simulink model "ASM_Traffic"  (R2026a)
settings: Solver=ode1  StartTime=SIM.tstart.v  StopTime=SIM.tend.v  FixedStep=SIM.StepSize.v
PostLoadFcn:
  | if any(exist('dsrtsu_mdlpostloadfcn', 'file') ~= 0), dsrtsu_mdlpostloadfcn('Execute', bdroot); end
  | try, asm_mdl_postloadfcn(bdroot, 'UpdateModel', 3600); catch, disp(lasterr); end,
InitFcn:
  | , if any(exist('rtifpga_mdlclblib', 'file') ~= 0), rtifpga_mdlclblib('Init', bdroot); end,
  | , if any(exist('dsmpb_private', 'file') ~= 0), dsmpb_private('dsmpb_mdlclblib', 'Init', bdroot); end,
model workspace (MAT data in the model file):
  asmReferencePath = [0 0.01 0.02 0.03 0.04 0.05 0.06 0.07 0.08 0.09 0.1 0.11 ... (350007 elements, 50001x7)]
  roadBounds : Simulink.Parameter (value not decoded)
  safetyAxes : Simulink.Parameter (value not decoded)
undefined symbols (not defined in the file): _to_, a0b2, ASM_BrakeHydraulics_DemoSystems, ASM_VehicleDynamics_DemoSystems, b98103fe8ad365046cd0, BrakeCircuit, controllerConfig, CPT, Crankshaft, DiscIntNeverNeededParam, dsmsi, FinalDriveAssembly, MDL, ModeSignals, mu, Pos_BrakePedal_Maneuver, rad, RefSignals, roadFamilyData, roadFamilyId, s_to_rpm, SIM, SoftECU, Suspension, Tire, Transmission
libraries: ASM_Traffic_lib x135, simulink x98, ASM_Utils_lib x77, ASM_VehicleDynamics_lib x70, ASM_Environment_lib x22, dsmpblib x20, dsmsilib x15, MDLD_Utils_lib x10, ASM_BrakeHydraulics_lib x3, sl_discontinuities x2
(part 53 of 65)

== system ASM_Traffic/Environment/Sensors/UserInterface/DISP_Plant/Object_Sensor_3D/IndexConflict_Info[] ==
  In1 : Inport
  Out1 : Outport  VectorParamsAs1DForOutWhenUnconnected=off
  wires:
  In1/1 -> Out1/1

== system ASM_Traffic/Environment/Sensors/UserInterface/DISP_Plant/Object_Sensor_3D/InputDataSamplePulse[0|1] ==
  In1 : Inport
  Out1 : Outport  VectorParamsAs1DForOutWhenUnconnected=off
  wires:
  In1/1 -> Out1/1

== system ASM_Traffic/Environment/Sensors/UserInterface/DISP_Plant/Object_Sensor_3D/Object_ID[] ==
  In1 : Inport
  Out1 : Outport  VectorParamsAs1DForOutWhenUnconnected=off
  wires:
  In1/1 -> Out1/1

== system ASM_Traffic/Environment/Sensors/UserInterface/DISP_Plant/Object_Sensor_3D/Object_ID[]1 ==
  In1 : Inport
  Out1 : Outport  VectorParamsAs1DForOutWhenUnconnected=off
  wires:
  In1/1 -> Out1/1

== system ASM_Traffic/Environment/Sensors/UserInterface/DISP_Plant/Object_Sensor_3D/Object_ID[]2 ==
  In1 : Inport
  Out1 : Outport  VectorParamsAs1DForOutWhenUnconnected=off
  wires:
  In1/1 -> Out1/1

== system ASM_Traffic/Environment/Sensors/UserInterface/DISP_Plant/Object_Sensor_3D/Object_Info[-1None|1Fellow|2Static] ==
  In1 : Inport
  Out1 : Outport  VectorParamsAs1DForOutWhenUnconnected=off
  wires:
  In1/1 -> Out1/1

== system ASM_Traffic/Environment/Sensors/UserInterface/DISP_Plant/Object_Sensor_3D/Object_Info[-1None|1Fellow|2Static]1 ==
  In1 : Inport
  Out1 : Outport  VectorParamsAs1DForOutWhenUnconnected=off
  wires:
  In1/1 -> Out1/1

== system ASM_Traffic/Environment/Sensors/UserInterface/DISP_Plant/Object_Sensor_3D/Object_Info[-1None|1Fellow|2Static]2 ==
  In1 : Inport
  Out1 : Outport  VectorParamsAs1DForOutWhenUnconnected=off
  wires:
  In1/1 -> Out1/1

== system ASM_Traffic/Environment/Sensors/UserInterface/DISP_Plant/Object_Sensor_3D/Object_Sensor_3D_VisualizationData ==
  TrafficBus : Inport
  Bus Selector1 : BusSelector  OutputSignals=Object_Sensor_3D.Sensor_1_Front_Long,Object_Sensor_3D.Sensor_2_Front_Mid,Object_Sensor_3D.Sensor_3_Rear
  Bus Selector2 : BusSelector  OutputSignals=Object_Sensor_3D.Sensor_1_Front_Long,Object_Sensor_3D.Sensor_2_Front_Mid,Object_Sensor_3D.Sensor_3_Rear
  Bus Selector9 : BusSelector  OutputSignals=Object_Sensor_3D.Sensor_1_Front_Long,Object_Sensor_3D.Sensor_2_Front_Mid,Object_Sensor_3D.Sensor_3_Rear
  Sensor_1_Front_Long_CustomPoints : Subsystem
  Sensor_1_Front_Long_NearestPoints : Subsystem
  Sensor_1_Front_Long_RadarReflectionPoints : Subsystem
  Sensor_2_Front_Mid_CustomPoints : Subsystem
  Sensor_2_Front_Mid_NearestPoints : Subsystem
  Sensor_2_Front_Mid_RadarReflectionPoints : Subsystem
  Sensor_3_Rear_CustomPoints : Subsystem
  Sensor_3_Rear_NearestPoints : Subsystem
  Sensor_3_Rear_RadarReflectionPoints : Subsystem
  wires:
  Bus Selector2/3 -> Sensor_3_Rear_CustomPoints/1(Sensor)  "<Sensor_3_Rear>"
  Bus Selector2/2 -> Sensor_2_Front_Mid_CustomPoints/1(Sensor)  "<Sensor_2_Front_Mid>"
  Bus Selector2/1 -> Sensor_1_Front_Long_CustomPoints/1(Sensor)  "<Sensor_1_Front_Long>"
  Bus Selector1/3 -> Sensor_3_Rear_RadarReflectionPoints/1(Sensor)  "<Sensor_3_Rear>"
  Bus Selector1/2 -> Sensor_2_Front_Mid_RadarReflectionPoints/1(Sensor)  "<Sensor_2_Front_Mid>"
  Bus Selector1/1 -> Sensor_1_Front_Long_RadarReflectionPoints/1(Sensor)  "<Sensor_1_Front_Long>"
  Bus Selector9/1 -> Sensor_1_Front_Long_NearestPoints/1(Sensor)  "<Sensor_1_Front_Long>"
  TrafficBus/1 -> Bus Selector9/1, Bus Selector1/1, Bus Selector2/1
  Bus Selector9/2 -> Sensor_2_Front_Mid_NearestPoints/1(Sensor)  "<Sensor_2_Front_Mid>"
  Bus Selector9/3 -> Sensor_3_Rear_NearestPoints/1(Sensor)  "<Sensor_3_Rear>"

== system ASM_Traffic/Environment/Sensors/UserInterface/DISP_Plant/Object_Sensor_3D/Object_Type[] ==
  In1 : Inport
  Out1 : Outport  VectorParamsAs1DForOutWhenUnconnected=off
  wires:
  In1/1 -> Out1/1

== system ASM_Traffic/Environment/Sensors/UserInterface/DISP_Plant/Object_Sensor_3D/Object_Type[]1 ==
  In1 : Inport
  Out1 : Outport  VectorParamsAs1DForOutWhenUnconnected=off
  wires:
  In1/1 -> Out1/1

== system ASM_Traffic/Environment/Sensors/UserInterface/DISP_Plant/Object_Sensor_3D/Object_Type[]2 ==
  In1 : Inport
  Out1 : Outport  VectorParamsAs1DForOutWhenUnconnected=off
  wires:
  In1/1 -> Out1/1

== system ASM_Traffic/Environment/Sensors/UserInterface/DISP_Plant/Object_Sensor_3D/Occlusion_Ratio_Object[-1|0_1] ==
  In1 : Inport
  Out1 : Outport  VectorParamsAs1DForOutWhenUnconnected=off
  wires:
  In1/1 -> Out1/1

== system ASM_Traffic/Environment/Sensors/UserInterface/DISP_Plant/Object_Sensor_3D/Occlusion_Ratio_Object[-1|0_1]1 ==
  In1 : Inport
  Out1 : Outport  VectorParamsAs1DForOutWhenUnconnected=off
  wires:
  In1/1 -> Out1/1

== system ASM_Traffic/Environment/Sensors/UserInterface/DISP_Plant/Object_Sensor_3D/Occlusion_Ratio_Object[-1|0_1]2 ==
  In1 : Inport
  Out1 : Outport  VectorParamsAs1DForOutWhenUnconnected=off
  wires:
  In1/1 -> Out1/1

== system ASM_Traffic/Environment/Sensors/UserInterface/DISP_Plant/Object_Sensor_3D/SensorEnable[0Off|1On] ==
  In1 : Inport
  Out1 : Outport  VectorParamsAs1DForOutWhenUnconnected=off
  wires:
  In1/1 -> Out1/1

== system ASM_Traffic/Environment/Sensors/UserInterface/DISP_Plant/Object_Sensor_3D/SensorIdx_Selected[] ==
  In1 : Inport
  Out1 : Outport  VectorParamsAs1DForOutWhenUnconnected=off
  wires:
  In1/1 -> Out1/1

== system ASM_Traffic/Environment/Sensors/UserInterface/DISP_Plant/Object_Sensor_3D/SensorSelection_Data[0|1] ==
  In1 : Inport
  Out1 : Outport  VectorParamsAs1DForOutWhenUnconnected=off
  wires:
  In1/1 -> Out1/1

== system ASM_Traffic/Environment/Sensors/UserInterface/DISP_Plant/Object_Sensor_3D/a_Rel_Object[m|s2] ==
  In1 : Inport
  Out1 : Outport  VectorParamsAs1DForOutWhenUnconnected=off
  wires:
  In1/1 -> Out1/1

== system ASM_Traffic/Environment/Sensors/UserInterface/DISP_Plant/Object_Sensor_3D/a_Rel_Object[m|s2]1 ==
  In1 : Inport
  Out1 : Outport  VectorParamsAs1DForOutWhenUnconnected=off
  wires:
  In1/1 -> Out1/1

== system ASM_Traffic/Environment/Sensors/UserInterface/DISP_Plant/Object_Sensor_3D/a_Rel_Object[m|s2]2 ==
  In1 : Inport
  Out1 : Outport  VectorParamsAs1DForOutWhenUnconnected=off
  wires:
  In1/1 -> Out1/1

== system ASM_Traffic/Environment/Sensors/UserInterface/DISP_Plant/Object_Sensor_3D/v_Rel_Object[m|s] ==
  In1 : Inport
  Out1 : Outport  VectorParamsAs1DForOutWhenUnconnected=off
  wires:
  In1/1 -> Out1/1

== system ASM_Traffic/Environment/Sensors/UserInterface/DISP_Plant/Object_Sensor_3D/v_Rel_Object[m|s]1 ==
  In1 : Inport
  Out1 : Outport  VectorParamsAs1DForOutWhenUnconnected=off
  wires:
  In1/1 -> Out1/1

== system ASM_Traffic/Environment/Sensors/UserInterface/DISP_Plant/Object_Sensor_3D/v_Rel_Object[m|s]2 ==
  In1 : Inport
  Out1 : Outport  VectorParamsAs1DForOutWhenUnconnected=off
  wires:
  In1/1 -> Out1/1

== system ASM_Traffic/Environment/Sensors/UserInterface/DISP_Plant/Traffic_Sign_Sensor/Angle_CoorSys_E[x;y;z][deg] ==
  In1 : Inport
  Out1 : Outport  VectorParamsAs1DForOutWhenUnconnected=off
  wires:
  In1/1 -> Out1/1

== system ASM_Traffic/Environment/Sensors/UserInterface/DISP_Plant/Traffic_Sign_Sensor/Angle_Hor_Rel[deg] ==
  In1 : Inport
  Out1 : Outport  VectorParamsAs1DForOutWhenUnconnected=off
  wires:
  In1/1 -> Out1/1

== system ASM_Traffic/Environment/Sensors/UserInterface/DISP_Plant/Traffic_Sign_Sensor/Angle_Ver_Rel[] ==
  In1 : Inport
  Out1 : Outport  VectorParamsAs1DForOutWhenUnconnected=off
  wires:
  In1/1 -> Out1/1

== system ASM_Traffic/Environment/Sensors/UserInterface/DISP_Plant/Traffic_Sign_Sensor/Distance[m] ==
  In1 : Inport
  Out1 : Outport  VectorParamsAs1DForOutWhenUnconnected=off
  wires:
  In1/1 -> Out1/1

== system ASM_Traffic/Environment/Sensors/UserInterface/DISP_Plant/Traffic_Sign_Sensor/GetTrfSgnDataByIndex_1 ==
  SelectSignDataByIndex : Inport
  TrafficBus : Inport  Port=2
  Saturation : Saturate  UpperLimit=MDL.Traffic.Sensors.TrafficSignSensorDyn_Calculation.Const_Sensor_Output_Dimension.v  LowerLimit=1
  SwitchObjectData : Subsystem
  SwitchObjectPosition : Subsystem
  SwitchSignProperties : Subsystem
  Traffic_Sign_Valid[0|1] : Outport  VectorParamsAs1DForOutWhenUnconnected=off
  TrafficObject_ID[] : Outport  Port=2  VectorParamsAs1DForOutWhenUnconnected=off
  TrafficObject_Type[] : Outport  Port=3  VectorParamsAs1DForOutWhenUnconnected=off
  Parent_Object_ID[] : Outport  Port=4  VectorParamsAs1DForOutWhenUnconnected=off
  Pos_CoorSys_E[x;y;z][m] : Outport  Port=5  VectorParamsAs1DForOutWhenUnconnected=off
  Angle_CoorSys_E[x;y;z][deg] : Outport  Port=6  VectorParamsAs1DForOutWhenUnconnected=off
  Pos_CoorSys_S[x;y;z][m] : Outport  Port=7  VectorParamsAs1DForOutWhenUnconnected=off
  Angle_Hor_Rel[deg] : Outport  Port=8  VectorParamsAs1DForOutWhenUnconnected=off
  Angle_Ver_Rel[deg] : Outport  Port=9  VectorParamsAs1DForOutWhenUnconnected=off
  Distance[m] : Outport  Port=10  VectorParamsAs1DForOutWhenUnconnected=off
  Traffic_Sign_Type[] : Outport  Port=11  VectorParamsAs1DForOutWhenUnconnected=off
  Traffic_Sign_Subtype[] : Outport  Port=12  VectorParamsAs1DForOutWhenUnconnected=off
  Traffic_Sign_Value[] : Outport  Port=13  VectorParamsAs1DForOutWhenUnconnected=off
  Traffic_Sign_Country[] : Outport  Port=14  VectorParamsAs1DForOutWhenUnconnected=off
  Traffic_Sign_Visibility[0_100] : Outport  Port=15  VectorParamsAs1DForOutWhenUnconnected=off
  Object_State[] : Outport  Port=16  VectorParamsAs1DForOutWhenUnconnected=off
  Object_Stream_ID[] : Outport  Port=17  VectorParamsAs1DForOutWhenUnconnected=off
  Traffic_Sign_Lanes[] : Outport  Port=18  VectorParamsAs1DForOutWhenUnconnected=off
  wires:
  SwitchSignProperties/8(Traffic_Sign_Lanes[]) -> Traffic_Sign_Lanes[]/1
  SwitchSignProperties/7(Object_Stream_ID[]) -> Object_Stream_ID[]/1
  SwitchSignProperties/6(Object_State[]) -> Object_State[]/1
  SwitchSignProperties/5(Traffic_Sign_Visibility[0_100]) -> Traffic_Sign_Visibility[0_100]/1
  SwitchSignProperties/4(Traffic_Sign_Country[]) -> Traffic_Sign_Country[]/1
  SwitchSignProperties/3(Traffic_Sign_Value[]) -> Traffic_Sign_Value[]/1
  SwitchSignProperties/2(Traffic_Sign_Subtype[]) -> Traffic_Sign_Subtype[]/1
  SwitchSignProperties/1(Traffic_Sign_Type[]) -> Traffic_Sign_Type[]/1
  SwitchObjectPosition/6(Distance[m]) -> Distance[m]/1
  SwitchObjectPosition/5(Angle_Ver_Rel[deg]) -> Angle_Ver_Rel[deg]/1
  SwitchObjectPosition/4(Angle_Hor_Rel[deg]) -> Angle_Hor_Rel[deg]/1
  SwitchObjectPosition/3(Pos_CoorSys_S[x;y;z][m]) -> Pos_CoorSys_S[x;y;z][m]/1
  SwitchObjectPosition/2(Angle_CoorSys_E[x;y;z][deg]) -> Angle_CoorSys_E[x;y;z][deg]/1
  SwitchObjectPosition/1(Pos_CoorSys_E[x;y;z][m]) -> Pos_CoorSys_E[x;y;z][m]/1
  SwitchObjectData/4(Parent_Object_ID[]) -> Parent_Object_ID[]/1
  SwitchObjectData/1(Traffic_Sign_Valid[0|1]) -> Traffic_Sign_Valid[0|1]/1
  SwitchObjectData/2(TrafficObject_ID[]) -> TrafficObject_ID[]/1
  TrafficBus/1 -> SwitchObjectData/1(TrafficBus), SwitchObjectPosition/1(TrafficBus), SwitchSignProperties/1(TrafficBus)
  SelectSignDataByIndex/1 -> Saturation/1
  SwitchObjectData/3(TrafficObject_Type[]) -> TrafficObject_Type[]/1
  Saturation/1 -> SwitchObjectData/2(Switch), SwitchObjectPosition/2(Switch), SwitchSignProperties/2(Switch)

== system ASM_Traffic/Environment/Sensors/UserInterface/DISP_Plant/Traffic_Sign_Sensor/Object_State[] ==
  In1 : Inport
  Out1 : Outport  VectorParamsAs1DForOutWhenUnconnected=off
  wires:
  In1/1 -> Out1/1

== system ASM_Traffic/Environment/Sensors/UserInterface/DISP_Plant/Traffic_Sign_Sensor/Object_Stream_ID[] ==
  In1 : Inport
  Out1 : Outport  VectorParamsAs1DForOutWhenUnconnected=off
  wires:
  In1/1 -> Out1/1

== system ASM_Traffic/Environment/Sensors/UserInterface/DISP_Plant/Traffic_Sign_Sensor/Parent_Object_ID[] ==
  In1 : Inport
  Out1 : Outport  VectorParamsAs1DForOutWhenUnconnected=off
  wires:
  In1/1 -> Out1/1

== system ASM_Traffic/Environment/Sensors/UserInterface/DISP_Plant/Traffic_Sign_Sensor/Pos_CoorSys_E[x;y;z][m] ==
  In1 : Inport
  Out1 : Outport  VectorParamsAs1DForOutWhenUnconnected=off
  wires:
  In1/1 -> Out1/1

== system ASM_Traffic/Environment/Sensors/UserInterface/DISP_Plant/Traffic_Sign_Sensor/Pos_CoorSys_S[x;y;z][m] ==
  In1 : Inport
  Out1 : Outport  VectorParamsAs1DForOutWhenUnconnected=off
  wires:
  In1/1 -> Out1/1

== system ASM_Traffic/Environment/Sensors/UserInterface/DISP_Plant/Traffic_Sign_Sensor/Sign_Valid[0|1] ==
  In1 : Inport
  Out1 : Outport  VectorParamsAs1DForOutWhenUnconnected=off
  wires:
  In1/1 -> Out1/1

== system ASM_Traffic/Environment/Sensors/UserInterface/DISP_Plant/Traffic_Sign_Sensor/TrafficObject_ID[] ==
  In1 : Inport
  Out1 : Outport  VectorParamsAs1DForOutWhenUnconnected=off
  wires:
  In1/1 -> Out1/1

== system ASM_Traffic/Environment/Sensors/UserInterface/DISP_Plant/Traffic_Sign_Sensor/TrafficObject_Type[] ==
  In1 : Inport
  Out1 : Outport  VectorParamsAs1DForOutWhenUnconnected=off
  wires:
  In1/1 -> Out1/1

== system ASM_Traffic/Environment/Sensors/UserInterface/DISP_Plant/Traffic_Sign_Sensor/TrafficSignSensor_Data_Valid[0|1] ==
  In1 : Inport
  Out1 : Outport  VectorParamsAs1DForOutWhenUnconnected=off
  wires:
  In1/1 -> Out1/1

== system ASM_Traffic/Environment/Sensors/UserInterface/DISP_Plant/Traffic_Sign_Sensor/TrafficSignSensor_Sfcn_State[] ==
  In1 : Inport
  Out1 : Outport  VectorParamsAs1DForOutWhenUnconnected=off
  wires:
  In1/1 -> Out1/1

== system ASM_Traffic/Environment/Sensors/UserInterface/DISP_Plant/Traffic_Sign_Sensor/Traffic_Sign_Country[] ==
  In1 : Inport
  Out1 : Outport  VectorParamsAs1DForOutWhenUnconnected=off
  wires:
  In1/1 -> Out1/1

== system ASM_Traffic/Environment/Sensors/UserInterface/DISP_Plant/Traffic_Sign_Sensor/Traffic_Sign_Lanes[] ==
  In1 : Inport
  Out1 : Outport  VectorParamsAs1DForOutWhenUnconnected=off
  wires:
  In1/1 -> Out1/1

== system ASM_Traffic/Environment/Sensors/UserInterface/DISP_Plant/Traffic_Sign_Sensor/Traffic_Sign_Subtype[] ==
  In1 : Inport
  Out1 : Outport  VectorParamsAs1DForOutWhenUnconnected=off
  wires:
  In1/1 -> Out1/1

== system ASM_Traffic/Environment/Sensors/UserInterface/DISP_Plant/Traffic_Sign_Sensor/Traffic_Sign_Type[] ==
  In1 : Inport
  Out1 : Outport  VectorParamsAs1DForOutWhenUnconnected=off
  wires:
  In1/1 -> Out1/1

== system ASM_Traffic/Environment/Sensors/UserInterface/DISP_Plant/Traffic_Sign_Sensor/Traffic_Sign_Value[] ==
  In1 : Inport
  Out1 : Outport  VectorParamsAs1DForOutWhenUnconnected=off
  wires:
  In1/1 -> Out1/1

== system ASM_Traffic/Environment/Sensors/UserInterface/DISP_Plant/Traffic_Sign_Sensor/Traffic_Sign_Visibility[0_100] ==
  In1 : Inport
  Out1 : Outport  VectorParamsAs1DForOutWhenUnconnected=off
  wires:
  In1/1 -> Out1/1

== system ASM_Traffic/Environment/Traffic/PlantModel/FellowMovement/ASMSignalBusCollect/avoid_incomplete_trace2source ==
  In1 : Inport
  DummyGain : Gain
  Out1 : Outport
  wires:
  DummyGain/1 -> Out1/1
  In1/1 -> DummyGain/1

== system ASM_Traffic/Environment/Traffic/PlantModel/FellowMovement/ASMSignalBusCollect/avoid_incomplete_trace2source1 ==
  In1 : Inport
  DummyGain : Gain
  Out1 : Outport
  wires:
  In1/1 -> DummyGain/1
  DummyGain/1 -> Out1/1

== system ASM_Traffic/Environment/Traffic/PlantModel/FellowMovement/ASMSignalBusCollect/avoid_incomplete_trace2source2 ==
  In1 : Inport
  DummyGain : Gain
  Out1 : Outport
  wires:
  DummyGain/1 -> Out1/1
  In1/1 -> DummyGain/1

== system ASM_Traffic/Environment/Traffic/PlantModel/FellowMovement/ASMSignalBusCollect/avoid_incomplete_trace2source3 ==
  In1 : Inport
  DummyGain : Gain
  Out1 : Outport
  wires:
  In1/1 -> DummyGain/1
  DummyGain/1 -> Out1/1

== system ASM_Traffic/Environment/Traffic/PlantModel/FellowMovement/LabelUserSignals/UserSignals_ ==
  UserSignals : Inport
  Demux : Demux  Outputs=10
      settings: DisplayOption=none
  User1[] : Outport  VectorParamsAs1DForOutWhenUnconnected=off
  User2[] : Outport  Port=2  VectorParamsAs1DForOutWhenUnconnected=off
  User3[] : Outport  Port=3  VectorParamsAs1DForOutWhenUnconnected=off
  User4[] : Outport  Port=4  VectorParamsAs1DForOutWhenUnconnected=off
  User5[] : Outport  Port=5  VectorParamsAs1DForOutWhenUnconnected=off
  User6[] : Outport  Port=6  VectorParamsAs1DForOutWhenUnconnected=off
  User7[] : Outport  Port=7  VectorParamsAs1DForOutWhenUnconnected=off
  User8[] : Outport  Port=8  VectorParamsAs1DForOutWhenUnconnected=off
  User9[] : Outport  Port=9  VectorParamsAs1DForOutWhenUnconnected=off
  User10[] : Outport  Port=10  VectorParamsAs1DForOutWhenUnconnected=off
  wires:
  UserSignals/1 -> Demux/1
  Demux/4 -> User4[]/1
  Demux/3 -> User3[]/1
  Demux/2 -> User2[]/1
  Demux/1 -> User1[]/1
  Demux/7 -> User7[]/1
  Demux/6 -> User6[]/1
  Demux/5 -> User5[]/1
  Demux/8 -> User8[]/1
  Demux/9 -> User9[]/1
  Demux/10 -> User10[]/1

== system ASM_Traffic/Environment/Traffic/PlantModel/FellowMovement/ObjectParameters_Modified/Yaw_Angle_Correction_Handling ==
  Movement_Characteristics[] : Inport
  Compare To Constant : simulink/Logic and Bit Operations/Compare To Constant  relop===  const=4  OutDataTypeStr=boolean
  use_yaw_road[0|1] : Outport
  wires:
  Movement_Characteristics[]/1 -> Compare To Constant/1
  Compare To Constant/1 -> use_yaw_road[0|1]/1

== system ASM_Traffic/Environment/Traffic/PlantModel/FellowMovement/Sw_SpeedLimit_Enable/SpeedLimit_RateLimiter ==
  In : Inport
  Gain : Gain  Gain=-1
  Multiport Switch : MultiPortSwitch  DataPortOrder=Zero-based contiguous  Inputs=2  DiagnosticForDefault=Warning  zeroidx=on  SaturateOnIntegerOverflow=off  InputSameDT=off
  Rate Limiter Dynamic : sl_discontinuities/Rate Limiter Dynamic
  RateLimit_ActivateThreshold[km|h] : simulink/Logic and Bit Operations/Compare To Constant  relop=>  const=200  OutDataTypeStr=uint8
  SpeedLimit_ChangeRate[km|h|s] : Constant  Value=20.0*ones(MDL.Traffic.MaxNumFellows.v,1)
  Unit Delay : UnitDelay  SampleTime=-1
  off : Constant  Value=1e8*ones(MDL.Traffic.MaxNumFellows.v,1)
  Out : Outport  VectorParamsAs1DForOutWhenUnconnected=off
  wires:
  Unit Delay/1 -> Rate Limiter Dynamic/1, Gain/1
  Rate Limiter Dynamic/1 -> Out/1
  In/1 -> RateLimit_ActivateThreshold[km|h]/1, Rate Limiter Dynamic/2
  Gain/1 -> Rate Limiter Dynamic/3
  Multiport Switch/1 -> Unit Delay/1
  SpeedLimit_ChangeRate[km|h|s]/1 -> Multiport Switch/2
  off/1 -> Multiport Switch/3
  RateLimit_ActivateThreshold[km|h]/1 -> Multiport Switch/1

== system ASM_Traffic/Environment/Traffic/PlantModel/Merge_Signals_toEnvironment/avoid_incomplete_trace2source/avoid_incomplete_trace2source ==
  In1 : Inport
  DummyGain : Gain
  Out1 : Outport
  wires:
  DummyGain/1 -> Out1/1
  In1/1 -> DummyGain/1

== system ASM_Traffic/Environment/Traffic/PlantModel/Merge_Signals_toEnvironment/avoid_incomplete_trace2source/avoid_incomplete_trace2source1 ==
  In1 : Inport
  DummyGain : Gain
  Out1 : Outport
  wires:
  In1/1 -> DummyGain/1
  DummyGain/1 -> Out1/1

== system ASM_Traffic/Environment/Traffic/PlantModel/Merge_Signals_toEnvironment/avoid_incomplete_trace2source/avoid_incomplete_trace2source2 ==
  In1 : Inport
  DummyGain : Gain
  Out1 : Outport
  wires:
  In1/1 -> DummyGain/1
  DummyGain/1 -> Out1/1

== system ASM_Traffic/Environment/Traffic/PlantModel/Merge_Signals_toEnvironment/avoid_incomplete_trace2source/avoid_incomplete_trace2source3 ==
  In1 : Inport
  DummyGain : Gain
  Out1 : Outport
  wires:
  DummyGain/1 -> Out1/1
  In1/1 -> DummyGain/1

== system ASM_Traffic/Environment/Traffic/PlantModel/Merge_Signals_toEnvironment/avoid_incomplete_trace2source/avoid_incomplete_trace2source4 ==
  In1 : Inport
  DummyGain : Gain
  Out1 : Outport
  wires:
  DummyGain/1 -> Out1/1
  In1/1 -> DummyGain/1

== system ASM_Traffic/Environment/Traffic/PlantModel/Merge_Signals_toEnvironment/avoid_incomplete_trace2source/avoid_incomplete_trace2source5 ==
  In1 : Inport
  DummyGain : Gain
  Out1 : Outport
  wires:
  In1/1 -> DummyGain/1
  DummyGain/1 -> Out1/1

== system ASM_Traffic/Environment/Traffic/UserInterface/DISP_Plant/Fellow_Movement/CurrentSegment[] ==
  In1 : Inport
  Out1 : Outport  VectorParamsAs1DForOutWhenUnconnected=off
  wires:
  In1/1 -> Out1/1

== system ASM_Traffic/Environment/Traffic/UserInterface/DISP_Plant/Fellow_Movement/CurrentSegment[]1 ==
  In1 : Inport
  Out1 : Outport  VectorParamsAs1DForOutWhenUnconnected=off
  wires:
  In1/1 -> Out1/1

== system ASM_Traffic/Environment/Traffic/UserInterface/DISP_Plant/Fellow_Movement/CurrentSegment[]2 ==
  In1 : Inport
  Out1 : Outport  VectorParamsAs1DForOutWhenUnconnected=off
  wires:
  In1/1 -> Out1/1

== system ASM_Traffic/Environment/Traffic/UserInterface/DISP_Plant/Fellow_Movement/CurrentSequence[] ==
  In1 : Inport
  Out1 : Outport  VectorParamsAs1DForOutWhenUnconnected=off
  wires:
  In1/1 -> Out1/1

== system ASM_Traffic/Environment/Traffic/UserInterface/DISP_Plant/Fellow_Movement/CurrentSequence[]1 ==
  In1 : Inport
  Out1 : Outport  VectorParamsAs1DForOutWhenUnconnected=off
  wires:
  In1/1 -> Out1/1

== system ASM_Traffic/Environment/Traffic/UserInterface/DISP_Plant/Fellow_Movement/CurrentSequence[]2 ==
  In1 : Inport
  Out1 : Outport  VectorParamsAs1DForOutWhenUnconnected=off
  wires:
  In1/1 -> Out1/1

== system ASM_Traffic/Environment/Traffic/UserInterface/DISP_Plant/Fellow_Movement/FlagFellowUsed[0|1] ==
  In1 : Inport
  Out1 : Outport  VectorParamsAs1DForOutWhenUnconnected=off
  wires:
  In1/1 -> Out1/1

== system ASM_Traffic/Environment/Traffic/UserInterface/DISP_Plant/Fellow_Movement/FlagFellowUsed[0|1]1 ==
  In1 : Inport
  Out1 : Outport  VectorParamsAs1DForOutWhenUnconnected=off
  wires:
  In1/1 -> Out1/1

== system ASM_Traffic/Environment/Traffic/UserInterface/DISP_Plant/Fellow_Movement/FlagFellowUsed[0|1]2 ==
  In1 : Inport
  Out1 : Outport  VectorParamsAs1DForOutWhenUnconnected=off
  wires:
  In1/1 -> Out1/1

== system ASM_Traffic/Environment/Traffic/UserInterface/DISP_Plant/Fellow_Movement/GetFellowDataByIndex_1 ==
  SelectFellowDataByIndex : Inport
  TrafficBus : Inport  Port=2
  Saturation : Saturate  UpperLimit=MDL.Traffic.MaxNumFellows.v  LowerLimit=1
  SwitchFellowMovementData : Subsystem
  SwitchInfoData : Subsystem
  CurrentSequence[] : Outport  VectorParamsAs1DForOutWhenUnconnected=off
  CurrentSegment[] : Outport  Port=2  VectorParamsAs1DForOutWhenUnconnected=off
  t_local[s] : Outport  Port=3  VectorParamsAs1DForOutWhenUnconnected=off
  FlagFellowUsed[0|1] : Outport  Port=4  VectorParamsAs1DForOutWhenUnconnected=off
  s_Fellow[m] : Outport  Port=5  VectorParamsAs1DForOutWhenUnconnected=off
  d_Total_Fellow[m] : Outport  Port=6  VectorParamsAs1DForOutWhenUnconnected=off
  v_Fellow[km|h] : Outport  Port=7  VectorParamsAs1DForOutWhenUnconnected=off
  wires:
  SwitchInfoData/1(CurrentSequence[]) -> CurrentSequence[]/1
  SwitchInfoData/2(CurrentSegment[]) -> CurrentSegment[]/1
  SwitchFellowMovementData/3("d_Total_Fellow[m] ") -> d_Total_Fellow[m]/1
  SwitchFellowMovementData/2("s_Fellow[m] ") -> s_Fellow[m]/1
  TrafficBus/1 -> SwitchFellowMovementData/1(TrafficBus), SwitchInfoData/1(TrafficBus)
  SelectFellowDataByIndex/1 -> Saturation/1
  SwitchFellowMovementData/4("v_Fellow[km|h] ") -> v_Fellow[km|h]/1
  SwitchFellowMovementData/1("Flag_Fellow_Used[0|1] ") -> FlagFellowUsed[0|1]/1
  SwitchInfoData/3(t_local[s]) -> t_local[s]/1
  Saturation/1 -> SwitchFellowMovementData/2(Switch), SwitchInfoData/2(Switch)

== system ASM_Traffic/Environment/Traffic/UserInterface/DISP_Plant/Fellow_Movement/GetFellowDataByIndex_2 ==
  SelectFellowDataByIndex : Inport
  TrafficBus : Inport  Port=2
  Saturation : Saturate  UpperLimit=MDL.Traffic.MaxNumFellows.v  LowerLimit=1
  SwitchFellowMovementData : Subsystem
  SwitchInfoData : Subsystem
  CurrentSequence[] : Outport  VectorParamsAs1DForOutWhenUnconnected=off
  CurrentSegment[] : Outport  Port=2  VectorParamsAs1DForOutWhenUnconnected=off
  t_local[s] : Outport  Port=3  VectorParamsAs1DForOutWhenUnconnected=off
  FlagFellowUsed[0|1] : Outport  Port=4  VectorParamsAs1DForOutWhenUnconnected=off
  s_Fellow[m] : Outport  Port=5  VectorParamsAs1DForOutWhenUnconnected=off
  d_Total_Fellow[m] : Outport  Port=6  VectorParamsAs1DForOutWhenUnconnected=off
  v_Fellow[km|h] : Outport  Port=7  VectorParamsAs1DForOutWhenUnconnected=off
  wires:
  SwitchInfoData/1(CurrentSequence[]) -> CurrentSequence[]/1
  SwitchInfoData/2(CurrentSegment[]) -> CurrentSegment[]/1
  SwitchFellowMovementData/3("d_Total_Fellow[m] ") -> d_Total_Fellow[m]/1
  SwitchFellowMovementData/2("s_Fellow[m] ") -> s_Fellow[m]/1
  TrafficBus/1 -> SwitchFellowMovementData/1(TrafficBus), SwitchInfoData/1(TrafficBus)
  SelectFellowDataByIndex/1 -> Saturation/1
  SwitchFellowMovementData/4("v_Fellow[km|h] ") -> v_Fellow[km|h]/1
  SwitchFellowMovementData/1("Flag_Fellow_Used[0|1] ") -> FlagFellowUsed[0|1]/1
  SwitchInfoData/3(t_local[s]) -> t_local[s]/1
  Saturation/1 -> SwitchFellowMovementData/2(Switch), SwitchInfoData/2(Switch)

== system ASM_Traffic/Environment/Traffic/UserInterface/DISP_Plant/Fellow_Movement/GetFellowDataByIndex_3 ==
  SelectFellowDataByIndex : Inport
  TrafficBus : Inport  Port=2
  Saturation : Saturate  UpperLimit=MDL.Traffic.MaxNumFellows.v  LowerLimit=1
  SwitchFellowMovementData : Subsystem
  SwitchInfoData : Subsystem
  CurrentSequence[] : Outport  VectorParamsAs1DForOutWhenUnconnected=off
  CurrentSegment[] : Outport  Port=2  VectorParamsAs1DForOutWhenUnconnected=off
  t_local[s] : Outport  Port=3  VectorParamsAs1DForOutWhenUnconnected=off
  FlagFellowUsed[0|1] : Outport  Port=4  VectorParamsAs1DForOutWhenUnconnected=off
  s_Fellow[m] : Outport  Port=5  VectorParamsAs1DForOutWhenUnconnected=off
  d_Total_Fellow[m] : Outport  Port=6  VectorParamsAs1DForOutWhenUnconnected=off
  v_Fellow[km|h] : Outport  Port=7  VectorParamsAs1DForOutWhenUnconnected=off
  wires:
  SwitchInfoData/1(CurrentSequence[]) -> CurrentSequence[]/1
  SwitchInfoData/2(CurrentSegment[]) -> CurrentSegment[]/1
  SwitchFellowMovementData/3("d_Total_Fellow[m] ") -> d_Total_Fellow[m]/1
  SwitchFellowMovementData/2("s_Fellow[m] ") -> s_Fellow[m]/1
  TrafficBus/1 -> SwitchFellowMovementData/1(TrafficBus), SwitchInfoData/1(TrafficBus)
  SelectFellowDataByIndex/1 -> Saturation/1
  SwitchFellowMovementData/4("v_Fellow[km|h] ") -> v_Fellow[km|h]/1
  SwitchFellowMovementData/1("Flag_Fellow_Used[0|1] ") -> FlagFellowUsed[0|1]/1
  SwitchInfoData/3(t_local[s]) -> t_local[s]/1
  Saturation/1 -> SwitchFellowMovementData/2(Switch), SwitchInfoData/2(Switch)

== system ASM_Traffic/Environment/Traffic/UserInterface/DISP_Plant/Fellow_Movement/d_Total_Fellow[m] ==
  In1 : Inport
  Out1 : Outport  VectorParamsAs1DForOutWhenUnconnected=off
  wires:
  In1/1 -> Out1/1

== system ASM_Traffic/Environment/Traffic/UserInterface/DISP_Plant/Fellow_Movement/d_Total_Fellow[m]1 ==
  In1 : Inport
  Out1 : Outport  VectorParamsAs1DForOutWhenUnconnected=off
  wires:
  In1/1 -> Out1/1

== system ASM_Traffic/Environment/Traffic/UserInterface/DISP_Plant/Fellow_Movement/d_Total_Fellow[m]2 ==
  In1 : Inport
  Out1 : Outport  VectorParamsAs1DForOutWhenUnconnected=off
  wires:
  In1/1 -> Out1/1

== system ASM_Traffic/Environment/Traffic/UserInterface/DISP_Plant/Fellow_Movement/s_Fellow[m] ==
  In1 : Inport
  Out1 : Outport  VectorParamsAs1DForOutWhenUnconnected=off
  wires:
  In1/1 -> Out1/1

== system ASM_Traffic/Environment/Traffic/UserInterface/DISP_Plant/Fellow_Movement/s_Fellow[m]1 ==
  In1 : Inport
  Out1 : Outport  VectorParamsAs1DForOutWhenUnconnected=off
  wires:
  In1/1 -> Out1/1

== system ASM_Traffic/Environment/Traffic/UserInterface/DISP_Plant/Fellow_Movement/s_Fellow[m]2 ==
  In1 : Inport
  Out1 : Outport  VectorParamsAs1DForOutWhenUnconnected=off
  wires:
  In1/1 -> Out1/1

== system ASM_Traffic/Environment/Traffic/UserInterface/DISP_Plant/Fellow_Movement/t_local[s] ==
  In1 : Inport
  Out1 : Outport  VectorParamsAs1DForOutWhenUnconnected=off
  wires:
  In1/1 -> Out1/1

== system ASM_Traffic/Environment/Traffic/UserInterface/DISP_Plant/Fellow_Movement/t_local[s]1 ==
  In1 : Inport
  Out1 : Outport  VectorParamsAs1DForOutWhenUnconnected=off
  wires:
  In1/1 -> Out1/1

== system ASM_Traffic/Environment/Traffic/UserInterface/DISP_Plant/Fellow_Movement/t_local[s]2 ==
  In1 : Inport
  Out1 : Outport  VectorParamsAs1DForOutWhenUnconnected=off
  wires:
  In1/1 -> Out1/1

== system ASM_Traffic/Environment/Traffic/UserInterface/DISP_Plant/Fellow_Movement/v_Fellow[km|h] ==
  In1 : Inport
  Out1 : Outport  VectorParamsAs1DForOutWhenUnconnected=off
  wires:
  In1/1 -> Out1/1

== system ASM_Traffic/Environment/Traffic/UserInterface/DISP_Plant/Fellow_Movement/v_Fellow[km|h]1 ==
  In1 : Inport
  Out1 : Outport  VectorParamsAs1DForOutWhenUnconnected=off
  wires:
  In1/1 -> Out1/1

== system ASM_Traffic/Environment/Traffic/UserInterface/DISP_Plant/Fellow_Movement/v_Fellow[km|h]2 ==
  In1 : Inport
  Out1 : Outport  VectorParamsAs1DForOutWhenUnconnected=off
  wires:
  In1/1 -> Out1/1

== system ASM_Traffic/Environment/Traffic/UserInterface/PAR_Plant/Fellow_Doors/Fellow10_Doors ==
  Bus Creator1 : BusCreator  Inputs=7
  SW_DoorFL[0Closed_1Open] : Constant  Value=0
  SW_DoorFR[0Closed_1Open] : Constant  Value=0
  SW_DoorRL[0Closed_1Open] : Constant  Value=0
  SW_DoorRR[0Closed_1Open] : Constant  Value=0
  SW_Hood[0Closed_1Open] : Constant  Value=0
  SW_ManualControl_Doors[1Scheduler|2Manual] : Constant
  SW_Trunk[0Closed_1Open] : Constant  Value=0
  Out1 : Outport  VectorParamsAs1DForOutWhenUnconnected=off
  wires:
  Bus Creator1/1 -> Out1/1
  SW_ManualControl_Doors[1Scheduler|2Manual]/1 -> Bus Creator1/1  "SW_ManualControl_Doors[1Scheduler|2Manual]"
  SW_DoorFL[0Closed_1Open]/1 -> Bus Creator1/2  "SW_DoorFL[0Closed_1Open]"
  SW_DoorFR[0Closed_1Open]/1 -> Bus Creator1/3  "SW_DoorFR[0Closed_1Open]"
  SW_DoorRL[0Closed_1Open]/1 -> Bus Creator1/4  "SW_DoorRL[0Closed_1Open]"
  SW_DoorRR[0Closed_1Open]/1 -> Bus Creator1/5  "SW_DoorRR[0Closed_1Open]"
  SW_Hood[0Closed_1Open]/1 -> Bus Creator1/6  "SW_Hood[0Closed_1Open]"
  SW_Trunk[0Closed_1Open]/1 -> Bus Creator1/7  "SW_Trunk[0Closed_1Open]"

== system ASM_Traffic/Environment/Traffic/UserInterface/PAR_Plant/Fellow_Doors/Fellow11_Doors ==
  Bus Creator1 : BusCreator  Inputs=7
  SW_DoorFL[0Closed_1Open] : Constant  Value=0
  SW_DoorFR[0Closed_1Open] : Constant  Value=0
  SW_DoorRL[0Closed_1Open] : Constant  Value=0
  SW_DoorRR[0Closed_1Open] : Constant  Value=0
  SW_Hood[0Closed_1Open] : Constant  Value=0
  SW_ManualControl_Doors[1Scheduler|2Manual] : Constant
  SW_Trunk[0Closed_1Open] : Constant  Value=0
  Out1 : Outport  VectorParamsAs1DForOutWhenUnconnected=off
  wires:
  Bus Creator1/1 -> Out1/1
  SW_ManualControl_Doors[1Scheduler|2Manual]/1 -> Bus Creator1/1  "SW_ManualControl_Doors[1Scheduler|2Manual]"
  SW_DoorFL[0Closed_1Open]/1 -> Bus Creator1/2  "SW_DoorFL[0Closed_1Open]"
  SW_DoorFR[0Closed_1Open]/1 -> Bus Creator1/3  "SW_DoorFR[0Closed_1Open]"
  SW_DoorRL[0Closed_1Open]/1 -> Bus Creator1/4  "SW_DoorRL[0Closed_1Open]"
  SW_DoorRR[0Closed_1Open]/1 -> Bus Creator1/5  "SW_DoorRR[0Closed_1Open]"
  SW_Hood[0Closed_1Open]/1 -> Bus Creator1/6  "SW_Hood[0Closed_1Open]"
  SW_Trunk[0Closed_1Open]/1 -> Bus Creator1/7  "SW_Trunk[0Closed_1Open]"

== system ASM_Traffic/Environment/Traffic/UserInterface/PAR_Plant/Fellow_Doors/Fellow12_Doors ==
  Bus Creator1 : BusCreator  Inputs=7
  SW_DoorFL[0Closed_1Open] : Constant  Value=0
  SW_DoorFR[0Closed_1Open] : Constant  Value=0
  SW_DoorRL[0Closed_1Open] : Constant  Value=0
  SW_DoorRR[0Closed_1Open] : Constant  Value=0
  SW_Hood[0Closed_1Open] : Constant  Value=0
  SW_ManualControl_Doors[1Scheduler|2Manual] : Constant
  SW_Trunk[0Closed_1Open] : Constant  Value=0
  Out1 : Outport  VectorParamsAs1DForOutWhenUnconnected=off
  wires:
  Bus Creator1/1 -> Out1/1
  SW_ManualControl_Doors[1Scheduler|2Manual]/1 -> Bus Creator1/1  "SW_ManualControl_Doors[1Scheduler|2Manual]"
  SW_DoorFL[0Closed_1Open]/1 -> Bus Creator1/2  "SW_DoorFL[0Closed_1Open]"
  SW_DoorFR[0Closed_1Open]/1 -> Bus Creator1/3  "SW_DoorFR[0Closed_1Open]"
  SW_DoorRL[0Closed_1Open]/1 -> Bus Creator1/4  "SW_DoorRL[0Closed_1Open]"
  SW_DoorRR[0Closed_1Open]/1 -> Bus Creator1/5  "SW_DoorRR[0Closed_1Open]"
  SW_Hood[0Closed_1Open]/1 -> Bus Creator1/6  "SW_Hood[0Closed_1Open]"
  SW_Trunk[0Closed_1Open]/1 -> Bus Creator1/7  "SW_Trunk[0Closed_1Open]"

== system ASM_Traffic/Environment/Traffic/UserInterface/PAR_Plant/Fellow_Doors/Fellow13_Doors ==
  Bus Creator1 : BusCreator  Inputs=7
  SW_DoorFL[0Closed_1Open] : Constant  Value=0
  SW_DoorFR[0Closed_1Open] : Constant  Value=0
  SW_DoorRL[0Closed_1Open] : Constant  Value=0
  SW_DoorRR[0Closed_1Open] : Constant  Value=0
  SW_Hood[0Closed_1Open] : Constant  Value=0
  SW_ManualControl_Doors[1Scheduler|2Manual] : Constant
  SW_Trunk[0Closed_1Open] : Constant  Value=0
  Out1 : Outport  VectorParamsAs1DForOutWhenUnconnected=off
  wires:
  Bus Creator1/1 -> Out1/1
  SW_ManualControl_Doors[1Scheduler|2Manual]/1 -> Bus Creator1/1  "SW_ManualControl_Doors[1Scheduler|2Manual]"
  SW_DoorFL[0Closed_1Open]/1 -> Bus Creator1/2  "SW_DoorFL[0Closed_1Open]"
  SW_DoorFR[0Closed_1Open]/1 -> Bus Creator1/3  "SW_DoorFR[0Closed_1Open]"
  SW_DoorRL[0Closed_1Open]/1 -> Bus Creator1/4  "SW_DoorRL[0Closed_1Open]"
  SW_DoorRR[0Closed_1Open]/1 -> Bus Creator1/5  "SW_DoorRR[0Closed_1Open]"
  SW_Hood[0Closed_1Open]/1 -> Bus Creator1/6  "SW_Hood[0Closed_1Open]"
  SW_Trunk[0Closed_1Open]/1 -> Bus Creator1/7  "SW_Trunk[0Closed_1Open]"

== system ASM_Traffic/Environment/Traffic/UserInterface/PAR_Plant/Fellow_Doors/Fellow14_Doors ==
  Bus Creator1 : BusCreator  Inputs=7
  SW_DoorFL[0Closed_1Open] : Constant  Value=0
  SW_DoorFR[0Closed_1Open] : Constant  Value=0
  SW_DoorRL[0Closed_1Open] : Constant  Value=0
  SW_DoorRR[0Closed_1Open] : Constant  Value=0
  SW_Hood[0Closed_1Open] : Constant  Value=0
  SW_ManualControl_Doors[1Scheduler|2Manual] : Constant
  SW_Trunk[0Closed_1Open] : Constant  Value=0
  Out1 : Outport  VectorParamsAs1DForOutWhenUnconnected=off
  wires:
  Bus Creator1/1 -> Out1/1
  SW_ManualControl_Doors[1Scheduler|2Manual]/1 -> Bus Creator1/1  "SW_ManualControl_Doors[1Scheduler|2Manual]"
  SW_DoorFL[0Closed_1Open]/1 -> Bus Creator1/2  "SW_DoorFL[0Closed_1Open]"
  SW_DoorFR[0Closed_1Open]/1 -> Bus Creator1/3  "SW_DoorFR[0Closed_1Open]"
  SW_DoorRL[0Closed_1Open]/1 -> Bus Creator1/4  "SW_DoorRL[0Closed_1Open]"
  SW_DoorRR[0Closed_1Open]/1 -> Bus Creator1/5  "SW_DoorRR[0Closed_1Open]"
  SW_Hood[0Closed_1Open]/1 -> Bus Creator1/6  "SW_Hood[0Closed_1Open]"
  SW_Trunk[0Closed_1Open]/1 -> Bus Creator1/7  "SW_Trunk[0Closed_1Open]"

== system ASM_Traffic/Environment/Traffic/UserInterface/PAR_Plant/Fellow_Doors/Fellow15_Doors ==
  Bus Creator1 : BusCreator  Inputs=7
  SW_DoorFL[0Closed_1Open] : Constant  Value=0
  SW_DoorFR[0Closed_1Open] : Constant  Value=0
  SW_DoorRL[0Closed_1Open] : Constant  Value=0
  SW_DoorRR[0Closed_1Open] : Constant  Value=0
  SW_Hood[0Closed_1Open] : Constant  Value=0
  SW_ManualControl_Doors[1Scheduler|2Manual] : Constant
  SW_Trunk[0Closed_1Open] : Constant  Value=0
  Out1 : Outport  VectorParamsAs1DForOutWhenUnconnected=off
  wires:
  Bus Creator1/1 -> Out1/1
  SW_ManualControl_Doors[1Scheduler|2Manual]/1 -> Bus Creator1/1  "SW_ManualControl_Doors[1Scheduler|2Manual]"
  SW_DoorFL[0Closed_1Open]/1 -> Bus Creator1/2  "SW_DoorFL[0Closed_1Open]"
  SW_DoorFR[0Closed_1Open]/1 -> Bus Creator1/3  "SW_DoorFR[0Closed_1Open]"
  SW_DoorRL[0Closed_1Open]/1 -> Bus Creator1/4  "SW_DoorRL[0Closed_1Open]"
  SW_DoorRR[0Closed_1Open]/1 -> Bus Creator1/5  "SW_DoorRR[0Closed_1Open]"
  SW_Hood[0Closed_1Open]/1 -> Bus Creator1/6  "SW_Hood[0Closed_1Open]"
  SW_Trunk[0Closed_1Open]/1 -> Bus Creator1/7  "SW_Trunk[0Closed_1Open]"

== system ASM_Traffic/Environment/Traffic/UserInterface/PAR_Plant/Fellow_Doors/Fellow16_Doors ==
  Bus Creator1 : BusCreator  Inputs=7
  SW_DoorFL[0Closed_1Open] : Constant  Value=0
  SW_DoorFR[0Closed_1Open] : Constant  Value=0
  SW_DoorRL[0Closed_1Open] : Constant  Value=0
  SW_DoorRR[0Closed_1Open] : Constant  Value=0
  SW_Hood[0Closed_1Open] : Constant  Value=0
  SW_ManualControl_Doors[1Scheduler|2Manual] : Constant
  SW_Trunk[0Closed_1Open] : Constant  Value=0
  Out1 : Outport  VectorParamsAs1DForOutWhenUnconnected=off
  wires:
  Bus Creator1/1 -> Out1/1
  SW_ManualControl_Doors[1Scheduler|2Manual]/1 -> Bus Creator1/1  "SW_ManualControl_Doors[1Scheduler|2Manual]"
  SW_DoorFL[0Closed_1Open]/1 -> Bus Creator1/2  "SW_DoorFL[0Closed_1Open]"
  SW_DoorFR[0Closed_1Open]/1 -> Bus Creator1/3  "SW_DoorFR[0Closed_1Open]"
  SW_DoorRL[0Closed_1Open]/1 -> Bus Creator1/4  "SW_DoorRL[0Closed_1Open]"
  SW_DoorRR[0Closed_1Open]/1 -> Bus Creator1/5  "SW_DoorRR[0Closed_1Open]"
  SW_Hood[0Closed_1Open]/1 -> Bus Creator1/6  "SW_Hood[0Closed_1Open]"
  SW_Trunk[0Closed_1Open]/1 -> Bus Creator1/7  "SW_Trunk[0Closed_1Open]"

== system ASM_Traffic/Environment/Traffic/UserInterface/PAR_Plant/Fellow_Doors/Fellow17_Doors ==
  Bus Creator1 : BusCreator  Inputs=7
  SW_DoorFL[0Closed_1Open] : Constant  Value=0
  SW_DoorFR[0Closed_1Open] : Constant  Value=0
  SW_DoorRL[0Closed_1Open] : Constant  Value=0
  SW_DoorRR[0Closed_1Open] : Constant  Value=0
  SW_Hood[0Closed_1Open] : Constant  Value=0
  SW_ManualControl_Doors[1Scheduler|2Manual] : Constant
  SW_Trunk[0Closed_1Open] : Constant  Value=0
  Out1 : Outport  VectorParamsAs1DForOutWhenUnconnected=off
  wires:
  Bus Creator1/1 -> Out1/1
  SW_ManualControl_Doors[1Scheduler|2Manual]/1 -> Bus Creator1/1  "SW_ManualControl_Doors[1Scheduler|2Manual]"
  SW_DoorFL[0Closed_1Open]/1 -> Bus Creator1/2  "SW_DoorFL[0Closed_1Open]"
  SW_DoorFR[0Closed_1Open]/1 -> Bus Creator1/3  "SW_DoorFR[0Closed_1Open]"
  SW_DoorRL[0Closed_1Open]/1 -> Bus Creator1/4  "SW_DoorRL[0Closed_1Open]"
  SW_DoorRR[0Closed_1Open]/1 -> Bus Creator1/5  "SW_DoorRR[0Closed_1Open]"
  SW_Hood[0Closed_1Open]/1 -> Bus Creator1/6  "SW_Hood[0Closed_1Open]"
  SW_Trunk[0Closed_1Open]/1 -> Bus Creator1/7  "SW_Trunk[0Closed_1Open]"

== system ASM_Traffic/Environment/Traffic/UserInterface/PAR_Plant/Fellow_Doors/Fellow18_Doors ==
  Bus Creator1 : BusCreator  Inputs=7
  SW_DoorFL[0Closed_1Open] : Constant  Value=0
  SW_DoorFR[0Closed_1Open] : Constant  Value=0
  SW_DoorRL[0Closed_1Open] : Constant  Value=0
  SW_DoorRR[0Closed_1Open] : Constant  Value=0
  SW_Hood[0Closed_1Open] : Constant  Value=0
  SW_ManualControl_Doors[1Scheduler|2Manual] : Constant
  SW_Trunk[0Closed_1Open] : Constant  Value=0
  Out1 : Outport  VectorParamsAs1DForOutWhenUnconnected=off
  wires:
  Bus Creator1/1 -> Out1/1
  SW_ManualControl_Doors[1Scheduler|2Manual]/1 -> Bus Creator1/1  "SW_ManualControl_Doors[1Scheduler|2Manual]"
  SW_DoorFL[0Closed_1Open]/1 -> Bus Creator1/2  "SW_DoorFL[0Closed_1Open]"
  SW_DoorFR[0Closed_1Open]/1 -> Bus Creator1/3  "SW_DoorFR[0Closed_1Open]"
  SW_DoorRL[0Closed_1Open]/1 -> Bus Creator1/4  "SW_DoorRL[0Closed_1Open]"
  SW_DoorRR[0Closed_1Open]/1 -> Bus Creator1/5  "SW_DoorRR[0Closed_1Open]"
  SW_Hood[0Closed_1Open]/1 -> Bus Creator1/6  "SW_Hood[0Closed_1Open]"
  SW_Trunk[0Closed_1Open]/1 -> Bus Creator1/7  "SW_Trunk[0Closed_1Open]"

== system ASM_Traffic/Environment/Traffic/UserInterface/PAR_Plant/Fellow_Doors/Fellow19_Doors ==
  Bus Creator1 : BusCreator  Inputs=7
  SW_DoorFL[0Closed_1Open] : Constant  Value=0
  SW_DoorFR[0Closed_1Open] : Constant  Value=0
  SW_DoorRL[0Closed_1Open] : Constant  Value=0
  SW_DoorRR[0Closed_1Open] : Constant  Value=0
  SW_Hood[0Closed_1Open] : Constant  Value=0
  SW_ManualControl_Doors[1Scheduler|2Manual] : Constant
  SW_Trunk[0Closed_1Open] : Constant  Value=0
  Out1 : Outport  VectorParamsAs1DForOutWhenUnconnected=off
  wires:
  Bus Creator1/1 -> Out1/1
  SW_ManualControl_Doors[1Scheduler|2Manual]/1 -> Bus Creator1/1  "SW_ManualControl_Doors[1Scheduler|2Manual]"
  SW_DoorFL[0Closed_1Open]/1 -> Bus Creator1/2  "SW_DoorFL[0Closed_1Open]"
  SW_DoorFR[0Closed_1Open]/1 -> Bus Creator1/3  "SW_DoorFR[0Closed_1Open]"
  SW_DoorRL[0Closed_1Open]/1 -> Bus Creator1/4  "SW_DoorRL[0Closed_1Open]"
  SW_DoorRR[0Closed_1Open]/1 -> Bus Creator1/5  "SW_DoorRR[0Closed_1Open]"
  SW_Hood[0Closed_1Open]/1 -> Bus Creator1/6  "SW_Hood[0Closed_1Open]"
  SW_Trunk[0Closed_1Open]/1 -> Bus Creator1/7  "SW_Trunk[0Closed_1Open]"

== system ASM_Traffic/Environment/Traffic/UserInterface/PAR_Plant/Fellow_Doors/Fellow1_Doors ==
  Bus Creator1 : BusCreator  Inputs=7
  SW_DoorFL[0Closed_1Open] : Constant  Value=0
  SW_DoorFR[0Closed_1Open] : Constant  Value=0
  SW_DoorRL[0Closed_1Open] : Constant  Value=0
  SW_DoorRR[0Closed_1Open] : Constant  Value=0
  SW_Hood[0Closed_1Open] : Constant  Value=0
  SW_ManualControl_Doors[1Scheduler|2Manual] : Constant
  SW_Trunk[0Closed_1Open] : Constant  Value=0
  Out1 : Outport  VectorParamsAs1DForOutWhenUnconnected=off
  wires:
  Bus Creator1/1 -> Out1/1
  SW_ManualControl_Doors[1Scheduler|2Manual]/1 -> Bus Creator1/1  "SW_ManualControl_Doors[1Scheduler|2Manual]"
  SW_DoorFL[0Closed_1Open]/1 -> Bus Creator1/2  "SW_DoorFL[0Closed_1Open]"
  SW_DoorFR[0Closed_1Open]/1 -> Bus Creator1/3  "SW_DoorFR[0Closed_1Open]"
  SW_DoorRL[0Closed_1Open]/1 -> Bus Creator1/4  "SW_DoorRL[0Closed_1Open]"
  SW_DoorRR[0Closed_1Open]/1 -> Bus Creator1/5  "SW_DoorRR[0Closed_1Open]"
  SW_Hood[0Closed_1Open]/1 -> Bus Creator1/6  "SW_Hood[0Closed_1Open]"
  SW_Trunk[0Closed_1Open]/1 -> Bus Creator1/7  "SW_Trunk[0Closed_1Open]"

== system ASM_Traffic/Environment/Traffic/UserInterface/PAR_Plant/Fellow_Doors/Fellow20_Doors ==
  Bus Creator1 : BusCreator  Inputs=7
  SW_DoorFL[0Closed_1Open] : Constant  Value=0
  SW_DoorFR[0Closed_1Open] : Constant  Value=0
  SW_DoorRL[0Closed_1Open] : Constant  Value=0
  SW_DoorRR[0Closed_1Open] : Constant  Value=0
  SW_Hood[0Closed_1Open] : Constant  Value=0
  SW_ManualControl_Doors[1Scheduler|2Manual] : Constant
  SW_Trunk[0Closed_1Open] : Constant  Value=0
  Out1 : Outport  VectorParamsAs1DForOutWhenUnconnected=off
  wires:
  Bus Creator1/1 -> Out1/1
  SW_ManualControl_Doors[1Scheduler|2Manual]/1 -> Bus Creator1/1  "SW_ManualControl_Doors[1Scheduler|2Manual]"
  SW_DoorFL[0Closed_1Open]/1 -> Bus Creator1/2  "SW_DoorFL[0Closed_1Open]"
  SW_DoorFR[0Closed_1Open]/1 -> Bus Creator1/3  "SW_DoorFR[0Closed_1Open]"
  SW_DoorRL[0Closed_1Open]/1 -> Bus Creator1/4  "SW_DoorRL[0Closed_1Open]"
  SW_DoorRR[0Closed_1Open]/1 -> Bus Creator1/5  "SW_DoorRR[0Closed_1Open]"
  SW_Hood[0Closed_1Open]/1 -> Bus Creator1/6  "SW_Hood[0Closed_1Open]"
  SW_Trunk[0Closed_1Open]/1 -> Bus Creator1/7  "SW_Trunk[0Closed_1Open]"

== system ASM_Traffic/Environment/Traffic/UserInterface/PAR_Plant/Fellow_Doors/Fellow21_Doors ==
  Bus Creator1 : BusCreator  Inputs=7
  SW_DoorFL[0Closed_1Open] : Constant  Value=0
  SW_DoorFR[0Closed_1Open] : Constant  Value=0
  SW_DoorRL[0Closed_1Open] : Constant  Value=0
  SW_DoorRR[0Closed_1Open] : Constant  Value=0
  SW_Hood[0Closed_1Open] : Constant  Value=0
  SW_ManualControl_Doors[1Scheduler|2Manual] : Constant
  SW_Trunk[0Closed_1Open] : Constant  Value=0
  Out1 : Outport  VectorParamsAs1DForOutWhenUnconnected=off
  wires:
  Bus Creator1/1 -> Out1/1
  SW_ManualControl_Doors[1Scheduler|2Manual]/1 -> Bus Creator1/1  "SW_ManualControl_Doors[1Scheduler|2Manual]"
  SW_DoorFL[0Closed_1Open]/1 -> Bus Creator1/2  "SW_DoorFL[0Closed_1Open]"
  SW_DoorFR[0Closed_1Open]/1 -> Bus Creator1/3  "SW_DoorFR[0Closed_1Open]"
  SW_DoorRL[0Closed_1Open]/1 -> Bus Creator1/4  "SW_DoorRL[0Closed_1Open]"
  SW_DoorRR[0Closed_1Open]/1 -> Bus Creator1/5  "SW_DoorRR[0Closed_1Open]"
  SW_Hood[0Closed_1Open]/1 -> Bus Creator1/6  "SW_Hood[0Closed_1Open]"
  SW_Trunk[0Closed_1Open]/1 -> Bus Creator1/7  "SW_Trunk[0Closed_1Open]"

== system ASM_Traffic/Environment/Traffic/UserInterface/PAR_Plant/Fellow_Doors/Fellow22_Doors ==
  Bus Creator1 : BusCreator  Inputs=7
  SW_DoorFL[0Closed_1Open] : Constant  Value=0
  SW_DoorFR[0Closed_1Open] : Constant  Value=0
  SW_DoorRL[0Closed_1Open] : Constant  Value=0
  SW_DoorRR[0Closed_1Open] : Constant  Value=0
  SW_Hood[0Closed_1Open] : Constant  Value=0
  SW_ManualControl_Doors[1Scheduler|2Manual] : Constant
  SW_Trunk[0Closed_1Open] : Constant  Value=0
  Out1 : Outport  VectorParamsAs1DForOutWhenUnconnected=off
  wires:
  Bus Creator1/1 -> Out1/1
  SW_ManualControl_Doors[1Scheduler|2Manual]/1 -> Bus Creator1/1  "SW_ManualControl_Doors[1Scheduler|2Manual]"
  SW_DoorFL[0Closed_1Open]/1 -> Bus Creator1/2  "SW_DoorFL[0Closed_1Open]"
  SW_DoorFR[0Closed_1Open]/1 -> Bus Creator1/3  "SW_DoorFR[0Closed_1Open]"
  SW_DoorRL[0Closed_1Open]/1 -> Bus Creator1/4  "SW_DoorRL[0Closed_1Open]"
  SW_DoorRR[0Closed_1Open]/1 -> Bus Creator1/5  "SW_DoorRR[0Closed_1Open]"
  SW_Hood[0Closed_1Open]/1 -> Bus Creator1/6  "SW_Hood[0Closed_1Open]"
  SW_Trunk[0Closed_1Open]/1 -> Bus Creator1/7  "SW_Trunk[0Closed_1Open]"

== system ASM_Traffic/Environment/Traffic/UserInterface/PAR_Plant/Fellow_Doors/Fellow23_Doors ==
  Bus Creator1 : BusCreator  Inputs=7
  SW_DoorFL[0Closed_1Open] : Constant  Value=0
  SW_DoorFR[0Closed_1Open] : Constant  Value=0
  SW_DoorRL[0Closed_1Open] : Constant  Value=0
  SW_DoorRR[0Closed_1Open] : Constant  Value=0
  SW_Hood[0Closed_1Open] : Constant  Value=0
  SW_ManualControl_Doors[1Scheduler|2Manual] : Constant
  SW_Trunk[0Closed_1Open] : Constant  Value=0
  Out1 : Outport  VectorParamsAs1DForOutWhenUnconnected=off
  wires:
  Bus Creator1/1 -> Out1/1
  SW_ManualControl_Doors[1Scheduler|2Manual]/1 -> Bus Creator1/1  "SW_ManualControl_Doors[1Scheduler|2Manual]"
  SW_DoorFL[0Closed_1Open]/1 -> Bus Creator1/2  "SW_DoorFL[0Closed_1Open]"
  SW_DoorFR[0Closed_1Open]/1 -> Bus Creator1/3  "SW_DoorFR[0Closed_1Open]"
  SW_DoorRL[0Closed_1Open]/1 -> Bus Creator1/4  "SW_DoorRL[0Closed_1Open]"
  SW_DoorRR[0Closed_1Open]/1 -> Bus Creator1/5  "SW_DoorRR[0Closed_1Open]"
  SW_Hood[0Closed_1Open]/1 -> Bus Creator1/6  "SW_Hood[0Closed_1Open]"
  SW_Trunk[0Closed_1Open]/1 -> Bus Creator1/7  "SW_Trunk[0Closed_1Open]"

== system ASM_Traffic/Environment/Traffic/UserInterface/PAR_Plant/Fellow_Doors/Fellow24_Doors ==
  Bus Creator1 : BusCreator  Inputs=7
  SW_DoorFL[0Closed_1Open] : Constant  Value=0
  SW_DoorFR[0Closed_1Open] : Constant  Value=0
  SW_DoorRL[0Closed_1Open] : Constant  Value=0
  SW_DoorRR[0Closed_1Open] : Constant  Value=0
  SW_Hood[0Closed_1Open] : Constant  Value=0
  SW_ManualControl_Doors[1Scheduler|2Manual] : Constant
  SW_Trunk[0Closed_1Open] : Constant  Value=0
  Out1 : Outport  VectorParamsAs1DForOutWhenUnconnected=off
  wires:
  Bus Creator1/1 -> Out1/1
  SW_ManualControl_Doors[1Scheduler|2Manual]/1 -> Bus Creator1/1  "SW_ManualControl_Doors[1Scheduler|2Manual]"
  SW_DoorFL[0Closed_1Open]/1 -> Bus Creator1/2  "SW_DoorFL[0Closed_1Open]"
  SW_DoorFR[0Closed_1Open]/1 -> Bus Creator1/3  "SW_DoorFR[0Closed_1Open]"
  SW_DoorRL[0Closed_1Open]/1 -> Bus Creator1/4  "SW_DoorRL[0Closed_1Open]"
  SW_DoorRR[0Closed_1Open]/1 -> Bus Creator1/5  "SW_DoorRR[0Closed_1Open]"
  SW_Hood[0Closed_1Open]/1 -> Bus Creator1/6  "SW_Hood[0Closed_1Open]"
  SW_Trunk[0Closed_1Open]/1 -> Bus Creator1/7  "SW_Trunk[0Closed_1Open]"

== system ASM_Traffic/Environment/Traffic/UserInterface/PAR_Plant/Fellow_Doors/Fellow25_Doors ==
  Bus Creator1 : BusCreator  Inputs=7
  SW_DoorFL[0Closed_1Open] : Constant  Value=0
  SW_DoorFR[0Closed_1Open] : Constant  Value=0
  SW_DoorRL[0Closed_1Open] : Constant  Value=0
  SW_DoorRR[0Closed_1Open] : Constant  Value=0
  SW_Hood[0Closed_1Open] : Constant  Value=0
  SW_ManualControl_Doors[1Scheduler|2Manual] : Constant
  SW_Trunk[0Closed_1Open] : Constant  Value=0
  Out1 : Outport  VectorParamsAs1DForOutWhenUnconnected=off
  wires:
  Bus Creator1/1 -> Out1/1
  SW_ManualControl_Doors[1Scheduler|2Manual]/1 -> Bus Creator1/1  "SW_ManualControl_Doors[1Scheduler|2Manual]"
  SW_DoorFL[0Closed_1Open]/1 -> Bus Creator1/2  "SW_DoorFL[0Closed_1Open]"
  SW_DoorFR[0Closed_1Open]/1 -> Bus Creator1/3  "SW_DoorFR[0Closed_1Open]"
  SW_DoorRL[0Closed_1Open]/1 -> Bus Creator1/4  "SW_DoorRL[0Closed_1Open]"
  SW_DoorRR[0Closed_1Open]/1 -> Bus Creator1/5  "SW_DoorRR[0Closed_1Open]"
  SW_Hood[0Closed_1Open]/1 -> Bus Creator1/6  "SW_Hood[0Closed_1Open]"
  SW_Trunk[0Closed_1Open]/1 -> Bus Creator1/7  "SW_Trunk[0Closed_1Open]"
